simulink model "My_gfm_battery_sil_1_Exciter_Dis"  (R2018b)
settings: Solver=ode23t  StartTime=0.0  StopTime=5  MaxStep=1e-4  RelTol=1e-3
PreLoadFcn:
  | modelDir = fileparts(get_param(bdroot,'FileName'));
  | 
  | load_system(fullfile(modelDir,'controls_element_lib.slx'));
  | load_system(fullfile(modelDir,'test_sequence_lib.slx'));
InitFcn:
  | close all;
  | clear all;
  | clc;
  | 
  | % frequency nominals
  | F_NOM = 60;
  | W_NOM = 2 * pi * F_NOM;
  | 
  | % base values relative to inverter
  | % --------------------------------
  | VLL_INV_NOM = 480;
  | P_INV_NOM = 1e6;
  | Q_INV_NOM = 0.5e6;
  | S_INV_NOM = sqrt(P_INV_NOM^2 + Q_INV_NOM^2);
  | 
  | I_INV_BASE = S_INV_NOM/(sqrt(3)*VLL_INV_NOM);
  | Z_INV_BASE = VLL_INV_NOM^2/S_INV_NOM;
  | L_INV_BASE = Z_INV_BASE / W_NOM;
  | C_INV_BASE = 1 / (Z_INV_BASE * W_NOM);
  | 
  | % nominal ratings for power system model
  | % --------------------------------------
  | INVERTER_COUNT = 100;
  | 
  | VLV_NOM = VLL_INV_NOM;
  | VMV_NOM = 35e3;
  | VHV_NOM = 230e3;
  | S_PLANT = INVERTER_COUNT * S_INV_NOM;
  | 
  | N_GSU = VHV_NOM/VMV_NOM;
  | N_MVT = VMV_NOM/VLV_NOM;
  | 
  | I_LV_BASE = S_PLANT/(sqrt(3)*VLV_NOM);
  | I_MV_BASE = S_PLANT/(sqrt(3)*VMV_NOM);
  | I_HV_BASE = S_PLANT/(sqrt(3)*VHV_NOM);
  | 
  | Z_LV_BASE = VLV_NOM^2/S_PLANT;
  | Z_MV_BASE = VMV_NOM^2/S_PLANT;
  | Z_HV_BASE = VHV_NOM^2/S_PLANT;
  | 
  | L_LV_BASE = Z_LV_BASE / W_NOM;
  | L_MV_BASE = Z_MV_BASE / W_NOM;
  | L_HV_BASE = Z_HV_BASE / W_NOM;
  | C_LV_BASE = 1 / (Z_LV_BASE * W_NOM);
  | C_MV_BASE = 1 / (Z_MV_BASE * W_NOM);
  | C_HV_BASE = 1 / (Z_HV_BASE * W_NOM);
undefined symbols (not defined in the file): D1, D11, Delta, DiscIntNeverNeededParam, gcbh, j, sps_rtmsupport, Ts
libraries: powerlib x70, simulink x29, test_sequence_lib x10, controls_element_lib x3, spsHalfBridgeModel x3
(part 6 of 6)

== system My_gfm_battery_sil_1_Exciter_Dis/My Inverter Controller /My_circuit_controls_A1/virtual damper/Damping HPF ==
  note: Forward integrator
  in : Inport
  Constant2 : Constant  Value=Ts
  Constant3 : Constant  Value=OmegaUp
  Constant4 : Constant  Value=OmegaDn
  Constant9 : Constant  Value=1/20000
  Delay : Delay  DelayLength=1  InitialCondition=0
  Gain : Gain  Gain=1/5
  Math Function : Math  Operator=reciprocal  SaturateOnIntegerOverflow=on
  MinMax : MinMax  Function=max  Inputs=2
  MinMax1 : MinMax  Inputs=2
  MinMax2 : MinMax  Inputs=2
  Product : Product
  Product1 : Product
  Product2 : Product
  Saturation : Saturate  UpperLimit=inf  LowerLimit=0
  Saturation1 : Saturate  UpperLimit=0  LowerLimit=-inf
  Sum : Sum  Inputs=|+-
  Sum1 : Sum  Inputs=|++
  Sum2 : Sum  Inputs=|++
  out : Outport
  wires:
  Gain/1 -> MinMax1/2, MinMax2/1
  [Ts] -> Product/1
  [Ts] -> Math Function/1
  Delay/1 -> Sum1/2, Sum/2
  MinMax1/1 -> [OmegaUp]
  Constant9/1 -> MinMax/2
  Sum/1 -> out/1, Product2/1, Product1/2
  Math Function/1 -> Gain/1
  Constant4/1 -> MinMax2/2
  Constant2/1 -> MinMax/1
  Saturation/1 -> Sum2/1
  Sum1/1 -> Delay/1
  Sum2/1 -> Product/2
  MinMax2/1 -> [OmegaDn]
  Product/1 -> Sum1/1
  [OmegaUp] -> Product1/1
  Constant3/1 -> MinMax1/1
  MinMax/1 -> [Ts]
  Product2/1 -> Saturation1/1
  in/1 -> Sum/1
  Product1/1 -> Saturation/1
  [OmegaDn] -> Product2/2
  Saturation1/1 -> Sum2/2

== system My_gfm_battery_sil_1_Exciter_Dis/My Inverter Controller /My_circuit_controls_A3/virtual damper/Damping HPF ==
  note: Forward integrator
  in : Inport
  Constant2 : Constant  Value=Ts
  Constant3 : Constant  Value=OmegaUp
  Constant4 : Constant  Value=OmegaDn
  Constant9 : Constant  Value=1/20000
  Delay : Delay  DelayLength=1  InitialCondition=0
  Gain : Gain  Gain=1/5
  Math Function : Math  Operator=reciprocal  SaturateOnIntegerOverflow=on
  MinMax : MinMax  Function=max  Inputs=2
  MinMax1 : MinMax  Inputs=2
  MinMax2 : MinMax  Inputs=2
  Product : Product
  Product1 : Product
  Product2 : Product
  Saturation : Saturate  UpperLimit=inf  LowerLimit=0
  Saturation1 : Saturate  UpperLimit=0  LowerLimit=-inf
  Sum : Sum  Inputs=|+-
  Sum1 : Sum  Inputs=|++
  Sum2 : Sum  Inputs=|++
  out : Outport
  wires:
  Gain/1 -> MinMax1/2, MinMax2/1
  [Ts] -> Product/1
  [Ts] -> Math Function/1
  Delay/1 -> Sum1/2, Sum/2
  MinMax1/1 -> [OmegaUp]
  Constant9/1 -> MinMax/2
  Sum/1 -> out/1, Product2/1, Product1/2
  Math Function/1 -> Gain/1
  Constant4/1 -> MinMax2/2
  Constant2/1 -> MinMax/1
  Saturation/1 -> Sum2/1
  Sum1/1 -> Delay/1
  Sum2/1 -> Product/2
  MinMax2/1 -> [OmegaDn]
  Product/1 -> Sum1/1
  [OmegaUp] -> Product1/1
  Constant3/1 -> MinMax1/1
  MinMax/1 -> [Ts]
  Product2/1 -> Saturation1/1
  in/1 -> Sum/1
  Product1/1 -> Saturation/1
  [OmegaDn] -> Product2/2
  Saturation1/1 -> Sum2/2

== system My_gfm_battery_sil_1_Exciter_Dis/My Inverter Controller /My_circuit_controls_A4/SOGI/Integrator1 ==
  In : Inport
  Ts : Inport  Port=2
  Delay1 : Delay  DelayLength=1
  Delay2 : Delay  DelayLength=1
  Delay3 : Delay  DelayLength=1
  Gain : Gain  Gain=1/12
  Gain1 : Gain  Gain=23
  Gain2 : Gain  Gain=16
  Gain3 : Gain  Gain=5
  Product : Product
  Sum : Sum  Inputs=|+-
  Sum1 : Sum  Inputs=|++
  Sum2 : Sum  Inputs=|++
  Out : Outport
  wires:
  Delay2/1 -> Gain2/1, Delay3/1
  Delay1/1 -> Sum2/2, Gain1/1, Delay2/1
  Delay3/1 -> Gain3/1
  Gain2/1 -> Sum/2
  Gain1/1 -> Sum/1
  Gain3/1 -> Sum1/2
  Sum/1 -> Sum1/1
  Gain/1 -> Sum2/1
  Sum2/1 -> Delay1/1
  Product/1 -> Gain/1
  Sum1/1 -> Out/1
  Ts/1 -> Product/2
  In/1 -> Product/1

== system My_gfm_battery_sil_1_Exciter_Dis/My Inverter Controller /My_circuit_controls_A4/SOGI/Integrator3 ==
  In : Inport
  Ts : Inport  Port=2
  Delay1 : Delay  DelayLength=1
  Delay2 : Delay  DelayLength=1
  Delay3 : Delay  DelayLength=1
  Gain : Gain  Gain=1/12
  Gain1 : Gain  Gain=23
  Gain2 : Gain  Gain=16
  Gain3 : Gain  Gain=5
  Product : Product
  Sum : Sum  Inputs=|+-
  Sum1 : Sum  Inputs=|++
  Sum2 : Sum  Inputs=|++
  Out : Outport
  wires:
  Delay2/1 -> Gain2/1, Delay3/1
  Delay1/1 -> Sum2/2, Gain1/1, Delay2/1
  Delay3/1 -> Gain3/1
  Gain2/1 -> Sum/2
  Gain1/1 -> Sum/1
  Gain3/1 -> Sum1/2
  Sum/1 -> Sum1/1
  Gain/1 -> Sum2/1
  Sum2/1 -> Delay1/1
  Product/1 -> Gain/1
  Sum1/1 -> Out/1
  Ts/1 -> Product/2
  In/1 -> Product/1

== system My_gfm_battery_sil_1_Exciter_Dis/My Inverter Controller /My_circuit_controls_A4/virtual damper/Damping HPF ==
  note: Forward integrator
  in : Inport
  Constant2 : Constant  Value=Ts
  Constant3 : Constant  Value=OmegaUp
  Constant4 : Constant  Value=OmegaDn
  Constant9 : Constant  Value=1/20000
  Delay : Delay  DelayLength=1  InitialCondition=0
  Gain : Gain  Gain=1/5
  Math Function : Math  Operator=reciprocal  SaturateOnIntegerOverflow=on
  MinMax : MinMax  Function=max  Inputs=2
  MinMax1 : MinMax  Inputs=2
  MinMax2 : MinMax  Inputs=2
  Product : Product
  Product1 : Product
  Product2 : Product
  Saturation : Saturate  UpperLimit=inf  LowerLimit=0
  Saturation1 : Saturate  UpperLimit=0  LowerLimit=-inf
  Sum : Sum  Inputs=|+-
  Sum1 : Sum  Inputs=|++
  Sum2 : Sum  Inputs=|++
  out : Outport
  wires:
  Gain/1 -> MinMax1/2, MinMax2/1
  [Ts] -> Product/1
  [Ts] -> Math Function/1
  Delay/1 -> Sum1/2, Sum/2
  MinMax1/1 -> [OmegaUp]
  Constant9/1 -> MinMax/2
  Sum/1 -> out/1, Product2/1, Product1/2
  Math Function/1 -> Gain/1
  Constant4/1 -> MinMax2/2
  Constant2/1 -> MinMax/1
  Saturation/1 -> Sum2/1
  Sum1/1 -> Delay/1
  Sum2/1 -> Product/2
  MinMax2/1 -> [OmegaDn]
  Product/1 -> Sum1/1
  [OmegaUp] -> Product1/1
  Constant3/1 -> MinMax1/1
  MinMax/1 -> [Ts]
  Product2/1 -> Saturation1/1
  in/1 -> Sum/1
  Product1/1 -> Saturation/1
  [OmegaDn] -> Product2/2
  Saturation1/1 -> Sum2/2

== system My_gfm_battery_sil_1_Exciter_Dis/My Inverter Controller /My_currentLimiting_B/Current_foldback1/LPF  ==
  In : Inport
  1/0.01 : Gain  Gain=1/0.01
  Integrator : Integrator
  Sum3 : Sum  Inputs=|+-
  Out : Outport  VectorParamsAs1DForOutWhenUnconnected=on
  wires:
  Integrator/1 -> Out/1, Sum3/2
  Sum3/1 -> 1/0.01/1
  In/1 -> Sum3/1
  1/0.01/1 -> Integrator/1

== system My_gfm_battery_sil_1_Exciter_Dis/My Inverter Controller /My_machineModel_Other Exciter/AVR/LPF ==
  In : Inport
  1/tauMeas : Gain  Gain=1/tauMeas
  Integrator : Integrator
  Sum3 : Sum  Inputs=|+-
  Out : Outport  VectorParamsAs1DForOutWhenUnconnected=on
  wires:
  Integrator/1 -> Out/1, Sum3/2
  Sum3/1 -> 1/tauMeas/1
  In/1 -> Sum3/1
  1/tauMeas/1 -> Integrator/1

== system My_gfm_battery_sil_1_Exciter_Dis/My Inverter Controller /My_machineModel_Other Exciter/AVR/V LPF ==
  In : Inport
  1/tpv : Gain  Gain=1/tpv
  Integrator : Integrator
  Sum3 : Sum  Inputs=|+-
  Out : Outport  VectorParamsAs1DForOutWhenUnconnected=on
  wires:
  Integrator/1 -> Out/1, Sum3/2
  Sum3/1 -> 1/tpv/1
  In/1 -> Sum3/1
  1/tpv/1 -> Integrator/1

== system My_gfm_battery_sil_1_Exciter_Dis/My Inverter Controller /My_machineModel_Other Exciter/AVR/assymmetric filter ==
  note: The saturation block is configured to cause a rapid rise, but much slow drop in output.
  in : Inport
  Gain1 : Gain  Gain=1/tauBkSt
  Integrator : Integrator
  Saturation1 : Saturate  UpperLimit=VllRated  LowerLimit=-0.02 * VllRated
  Sum3 : Sum  Inputs=|+-
  out : Outport  VectorParamsAs1DForOutWhenUnconnected=on
  wires:
  Saturation1/1 -> Integrator/1
  Gain1/1 -> Saturation1/1
  in/1 -> Sum3/1
  Sum3/1 -> Gain1/1
  Integrator/1 -> Sum3/2, out/1

== system My_gfm_battery_sil_1_Exciter_Dis/My Inverter Controller /My_machineModel_Other Exciter/Exciter/LPF ==
  In : Inport
  Integrator : Integrator
  Sum3 : Sum  Inputs=|+-
  wExciter : Gain  Gain=wExciter
  Out : Outport  VectorParamsAs1DForOutWhenUnconnected=on
  wires:
  Integrator/1 -> Out/1, Sum3/2
  Sum3/1 -> wExciter/1
  In/1 -> Sum3/1
  wExciter/1 -> Integrator/1

== system My_gfm_battery_sil_1_Exciter_Dis/My Inverter Controller /My_machineModel_Other Exciter/Exciter/modulator ==
  cmd : Inport
  osc : Inport  Port=2
  Complex to Real-Imag : ComplexToRealImag
  Complex to Real-Imag1 : ComplexToRealImag
  Gain : Gain  Gain=sqrt(2)
  Product1 : Product
  Product2 : Product
  Sum1 : Sum  Inputs=|+-
  ref : Outport  VectorParamsAs1DForOutWhenUnconnected=on
  wires:
  osc/1 -> Gain/1
  Complex to Real-Imag/1 -> Product2/2
  Product2/1 -> Sum1/1
  Sum1/1 -> ref/1  "i"
  Gain/1 -> Complex to Real-Imag/1
  Complex to Real-Imag/2 -> Product1/2
  Product1/1 -> Sum1/2
  cmd/1 -> Complex to Real-Imag1/1
  Complex to Real-Imag1/1 -> Product2/1
  Complex to Real-Imag1/2 -> Product1/1

== system My_gfm_battery_sil_1_Exciter_Dis/My Inverter Controller /My_machineModel_Other Exciter/governer/LPF(DamperDecoupler) limited  ==
  In : Inport
  Constant : Constant  Value=1/tau_damp
  Constant1 : Constant  Value=wGoverner
  Integrator : Integrator  LimitOutput=on  UpperSaturationLimit=1.2*SRated  LowerSaturationLimit=-1.2*SRated
  MinMax : MinMax  Inputs=2
  Product : Product
  Sum3 : Sum  Inputs=|+-
  Out : Outport  VectorParamsAs1DForOutWhenUnconnected=on
  wires:
  Integrator/1 -> Out/1, Sum3/2
  Sum3/1 -> Product/2
  In/1 -> Sum3/1
  Product/1 -> Integrator/1
  MinMax/1 -> Product/1
  Constant/1 -> MinMax/1
  Constant1/1 -> MinMax/2

== system My_gfm_battery_sil_1_Exciter_Dis/My Inverter Controller /My_machineModel_Other Exciter/governer/synchronizer ==
  note: Big Range?
  note: prevent it from acting during typical faults
  note: Prevent loss of sync at low voltage events, using asym filter to traget long extended low voltage events
  note: Keeps the machine spining in synchronize while machine is disabled, disabling the machine means
  note: Why?
  Vq : Inport
  Vt : Inport  Port=2
  machine_enabled : Inport  Port=3
  Constant : Constant
  Gain : Gain  Gain=SRated
  Gain2 : Gain  Gain=1/VllRated
  "HPF " : Subsystem
  Product1 : Product
  Saturation : Saturate  UpperLimit=1  LowerLimit=0
  Sum : Sum  Inputs=|++
  Sum2 : Sum  Inputs=|+-
  Switch : Switch  Criteria=u2 > Threshold
  assymmetric filter1 : Subsystem
  gain : Gain  Gain=wSync
  kFastSync : Gain  Gain=kpFastSync
  kSync : Gain  Gain=kpSync
  pSyncLimit : Saturate  UpperLimit=3  LowerLimit=-3
  syncFadeGain : Gain  Gain=kpSyncFade
  syncFadeThreshold : Constant  Value=SyncFadeThres
  to_pu : Gain  Gain=1 / VllRated
  p_sync_pu : Outport  VectorParamsAs1DForOutWhenUnconnected=on
  wires:
  to_pu/1 -> Sum2/2
  Vt/1 -> assymmetric filter1/1(in)
  assymmetric filter1/1(out) -> to_pu/1
  pSyncLimit/1 -> Gain/1
  kSync/1 -> Sum/1
  Sum/1 -> pSyncLimit/1
  Product1/1 -> p_sync_pu/1
  Constant/1 -> Switch/3
  Sum2/1 -> syncFadeGain/1
  machine_enabled/1 -> Switch/2
  syncFadeGain/1 -> Saturation/1
  Saturation/1 -> Switch/1
  syncFadeThreshold/1 -> Sum2/1
  Switch/1 -> Product1/2
  Gain2/1 -> kFastSync/1, kSync/1
  Vq/1 -> Gain2/1
  Gain/1 -> Product1/1  "p_sync"
  kFastSync/1 -> "HPF "/1(in)
  "HPF "/1(out) -> gain/1
  gain/1 -> Sum/2

== system My_gfm_battery_sil_1_Exciter_Dis/My Inverter Controller /My_machineModel_Other Exciter/rotor model/HPF (wDamperDecoupler) 1 ==
  in : Inport
  1/tau_damp : Gain  Gain=1/tau_damp
  Integrator : Integrator
  Sum : Sum  Inputs=|+-
  out : Outport  VectorParamsAs1DForOutWhenUnconnected=on
  wires:
  Sum/1 -> out/1, 1/tau_damp/1
  in/1 -> Sum/1
  Integrator/1 -> Sum/2
  1/tau_damp/1 -> Integrator/1

== system My_gfm_battery_sil_1_Exciter_Dis/My Inverter Controller /My_machineModel_Other Exciter/rotor model/oscillator_3ph ==
  f : Inport
  Cos : Trigonometry  Operator=cos
  Gain : Gain  Gain=2*pi
  Integrator : Integrator
  Real-Imag to Complex : RealImagToComplex
  Sin : Trigonometry
  Sum1 : Sum  Inputs=|++
  phase_shift : Constant  Value=[0 -1/3 -2/3]
  osc[3] : Outport  VectorParamsAs1DForOutWhenUnconnected=on
  wires:
  f/1 -> Integrator/1
  Real-Imag to Complex/1 -> osc[3]/1
  Cos/1 -> Real-Imag to Complex/1
  Gain/1 -> Cos/1, Sin/1
  Integrator/1 -> Sum1/1
  Sin/1 -> Real-Imag to Complex/2
  phase_shift/1 -> Sum1/2
  Sum1/1 -> Gain/1

== system My_gfm_battery_sil_1_Exciter_Dis/My Inverter Controller /My_machineModel_Other Exciter/voltage analyzer/LPF ==
  In : Inport
  1/tauMeas : Gain  Gain=1/tauMeas
  Integrator : Integrator
  Sum3 : Sum  Inputs=|+-
  Out : Outport  VectorParamsAs1DForOutWhenUnconnected=on
  wires:
  Integrator/1 -> Out/1, Sum3/2
  Sum3/1 -> 1/tauMeas/1
  In/1 -> Sum3/1
  1/tauMeas/1 -> Integrator/1

== system My_gfm_battery_sil_1_Exciter_Dis/My Inverter Controller /My_machineModel_Other Exciter/voltage analyzer/LPF  ==
  In : Inport
  1/tauMeas : Gain  Gain=1/tauMeas
  Integrator : Integrator
  Sum3 : Sum  Inputs=|+-
  Out : Outport  VectorParamsAs1DForOutWhenUnconnected=on
  wires:
  Integrator/1 -> Out/1, Sum3/2
  Sum3/1 -> 1/tauMeas/1
  In/1 -> Sum3/1
  1/tauMeas/1 -> Integrator/1

== system My_gfm_battery_sil_1_Exciter_Dis/Plant controller (simplified example)/Meter/PLL-analog/oscillator_3ph ==
  f : Inport
  Cos : Trigonometry  Operator=cos
  Gain : Gain  Gain=2*pi
  Integrator : Integrator
  Real-Imag to Complex : RealImagToComplex
  Sin : Trigonometry
  Sum1 : Sum  Inputs=|++
  phase_shift : Constant  Value=[0 -1/3 -2/3]
  osc[3] : Outport  VectorParamsAs1DForOutWhenUnconnected=on
  wires:
  Sum1/1 -> Gain/1
  phase_shift/1 -> Sum1/2
  Sin/1 -> Real-Imag to Complex/2
  Integrator/1 -> Sum1/1
  Gain/1 -> Sin/1, Cos/1
  Cos/1 -> Real-Imag to Complex/1
  Real-Imag to Complex/1 -> osc[3]/1
  f/1 -> Integrator/1

== system My_gfm_battery_sil_1_Exciter_Dis/My Inverter Controller /My_machineModel_Other Exciter/governer/synchronizer/HPF  ==
  in : Inport
  Integrator : Integrator
  Sum : Sum  Inputs=|+-
  wSync : Gain  Gain=wSync
  out : Outport  VectorParamsAs1DForOutWhenUnconnected=on
  wires:
  Sum/1 -> out/1, wSync/1
  in/1 -> Sum/1
  Integrator/1 -> Sum/2
  wSync/1 -> Integrator/1

== system My_gfm_battery_sil_1_Exciter_Dis/My Inverter Controller /My_machineModel_Other Exciter/governer/synchronizer/assymmetric filter1 ==
  note: The saturation block is configured to cause a rapid rise, but much slow drop in output.
  in : Inport
  Gain1 : Gain  Gain=1/tauBkSt
  Integrator : Integrator
  Saturation1 : Saturate  UpperLimit=VllRated  LowerLimit=-0.02 * VllRated
  Sum3 : Sum  Inputs=|+-
  out : Outport  VectorParamsAs1DForOutWhenUnconnected=on
  wires:
  Integrator/1 -> out/1, Sum3/2
  Sum3/1 -> Gain1/1
  in/1 -> Sum3/1
  Gain1/1 -> Saturation1/1
  Saturation1/1 -> Integrator/1

== matlab function My_gfm_battery_sil_1_Exciter_Dis/ac Network with MVT (native math)5/Two-Level Converter/Model1/MATLAB Function ==
  data: g input; V output; Vdc input; I input; Idc output
function [V,Idc] = FunctionHalfBridge1(g,Vdc,I)
[V,Idc]=FunctionHalfBridge(g,Vdc,I);

== matlab function My_gfm_battery_sil_1_Exciter_Dis/ac Network with MVT (native math)5/Two-Level Converter/Model2/MATLAB Function ==
  data: g input; V output; Vdc input; I input; Idc output
function [V,Idc] = FunctionHalfBridge1(g,Vdc,I)
[V,Idc]=FunctionHalfBridge(g,Vdc,I);

== matlab function My_gfm_battery_sil_1_Exciter_Dis/ac Network with MVT (native math)5/Two-Level Converter/Model3/MATLAB Function ==
  data: g input; V output; Vdc input; I input; Idc output
function [V,Idc] = FunctionHalfBridge1(g,Vdc,I)
[V,Idc]=FunctionHalfBridge(g,Vdc,I);
